simulink model "LQR_CanBang"  (R2024b)
settings: Solver=FixedStepDiscrete  StartTime=0.0  StopTime=12  FixedStep=0.0050000000000000001  RelTol=1e-3
InitFcn:
  | addpath(fullfile(fileparts(fileparts(get_param(bdroot,'FileName'))),'shared'));
model workspace (MAT data in the model file):
  cfg.schema_version = 1
  cfg.config_id = 'nema17-relative-v1'
  cfg.hardware_confirmed = 0
  cfg.model.mb = 1.141
  cfg.model.mw = 0.033
  cfg.model.r = 0.033
  cfg.model.l = 0.035
  cfg.model.h = 0.14
  cfg.model.W = 0.228
  cfg.model.Ir = 3.6e-06
  cfg.model.g = 9.81
  cfg.drive.full_steps = 200
  cfg.drive.microstep = 16
  cfg.drive.max_relative_speed = 0.6
  cfg.drive.max_relative_accel = 3
  cfg.drive.max_step_hz = 15000
  cfg.drive.assumed_torque_per_motor = 0.08
  cfg.timing.lqr_s = 0.005
  cfg.timing.pid_s = 0.02
  cfg.timing.telemetry_s = 0.04
  cfg.timing.lease_s = 0.4
  cfg.timing.imu_max_age_s = 0.015
  cfg.timing.stable_s = 1
  cfg.lqr.state_order = {'theta_rad'; 'omega_rad_s'}
  cfg.lqr.input = 'relative_tangential_acceleration_m_s2'
  cfg.lqr.baseline_Q = [25; 1]
  cfg.lqr.baseline_R = 2
  cfg.lqr.Q = [400; 4]
  cfg.lqr.R = 1
  cfg.pid.velocity.kp = 1.2
  cfg.pid.velocity.ki = 0.25
  cfg.pid.velocity.kd = 0.04
  cfg.pid.yaw.kp = 3
  cfg.pid.yaw.ki = 0.8
  cfg.pid.yaw.kd = 0.02
  cfg.pid.derivative_tau_s = 0.08
  cfg.pid.accel_filter_s = 0.12
  cfg.pid.accel_max = 0.35
  cfg.pid.yaw_accel_max = 2
  cfg.pid.velocity_max = 0.2
  cfg.pid.yaw_rate_max = 0.8
  cfg.pid.velocity_slew = 0.12
  cfg.pid.yaw_slew = 0.6
  cfg.safety.arm_rad = 0.0698131700798
  cfg.safety.fall_rad = 0.383972435439
  cfg.safety.stable_rad = 0.0523598775598
  cfg.safety.stable_rate = 0.15
  cfg.safety.arm_rate = 0.3
  cfg.safety.arm_s = 1
  cfg.safety.deadline_fault_s = 0.015
  cfg.safety.saturation_fault_s = 0.3
  cfg.provisional_ranges.mb = [0.9; 1.4]
  cfg.provisional_ranges.mw = [0.0165; 0.033]
  cfg.provisional_ranges.r = [0.033; 0.04]
  cfg.provisional_ranges.l = [0.025; 0.06]
  cfg.provisional_ranges.Jc_scale = [0.6; 1.5]
  cfg.provisional_ranges.W = [0.16; 0.228]
  cfg.provisional_ranges.actuator_delay_s = [0; 0.005; 0.01]
  cfg.provisional_ranges.tracking_gain = [0.8; 1; 1.2]
  gain = [-23.7933968348 -2.75423353981]
  initial_state = [0.0872664625997; 0; 0; 0; 0; 0]
  reference_input = [0  0  0  0  1  0; 12  0  0  0  1  0]
settings Model: Creator=SON TUNG  LastModifiedBy=SON TUNG
settings DataIOCC: SaveOutput=off  SignalLogging=off

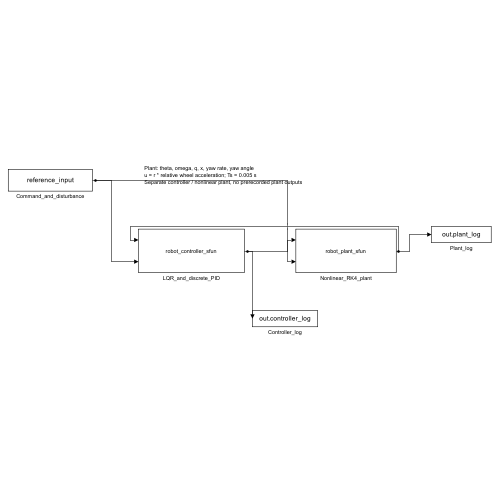
[thumbnail: Simulink's stored preview of the top-level diagram]
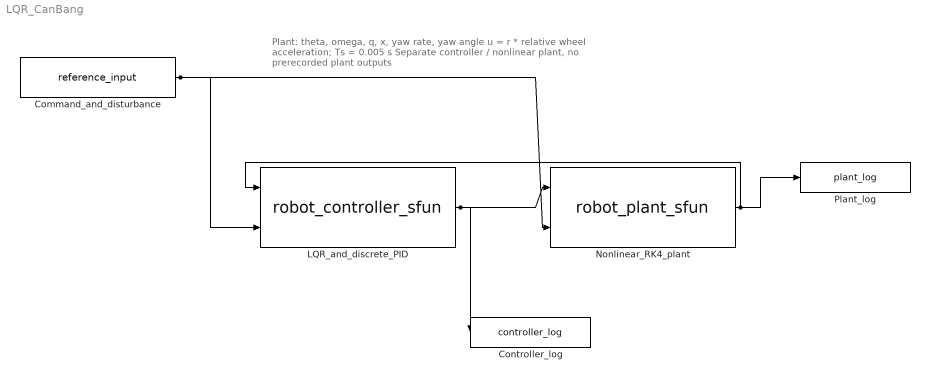
== system LQR_CanBang ==
  note: Plant: theta, omega, q, x, yaw rate, yaw angle
      | u = r * relative wheel acceleration; Ts = 0.005 s
      | Separate controller / nonlinear plant, no prerecorded plant outputs
  Command_and_disturbance : FromWorkspace  VariableName=reference_input  Interpolate=off  OutputAfterFinalValue=Holding final value
  Controller_log : ToWorkspace  VariableName=controller_log  SaveFormat=Timeseries  SampleTime=-1
  LQR_and_discrete_PID : M-S-Function  FunctionName=robot_controller_sfun  Parameters=cfg,gain
  Nonlinear_RK4_plant : M-S-Function  FunctionName=robot_plant_sfun  Parameters=cfg,initial_state
  Plant_log : ToWorkspace  VariableName=plant_log  SaveFormat=Timeseries  SampleTime=-1
  wires:
  Command_and_disturbance/1 -> LQR_and_discrete_PID/2, Nonlinear_RK4_plant/2
  LQR_and_discrete_PID/1 -> Nonlinear_RK4_plant/1, Controller_log/1
  Nonlinear_RK4_plant/1 -> LQR_and_discrete_PID/1, Plant_log/1
